simulink model "six_pulse_thyristor_based_rectifier"  (R2026b)
settings: Solver=ode23tb  StopTime=param.sim.simlength  FixedStep=param.glb_time.tc  MaxStep=param.glb_time.tc  EnableMultiTasking=on
values from neighbouring files (symbols this model uses):
  param = struct()    [init_model.m]    (also in init_model_legacy.m = add_template_extras(param, options))
undefined symbols (not defined in the file or in its folder): magnitude
libraries: fl_lib x168, nesl_utility x52, ee_lib x8, thyristor_rr_lib x6, first_harmonic_tracker x3, three_phase_voltage_with_frt_emulator x1
(part 2 of 4)

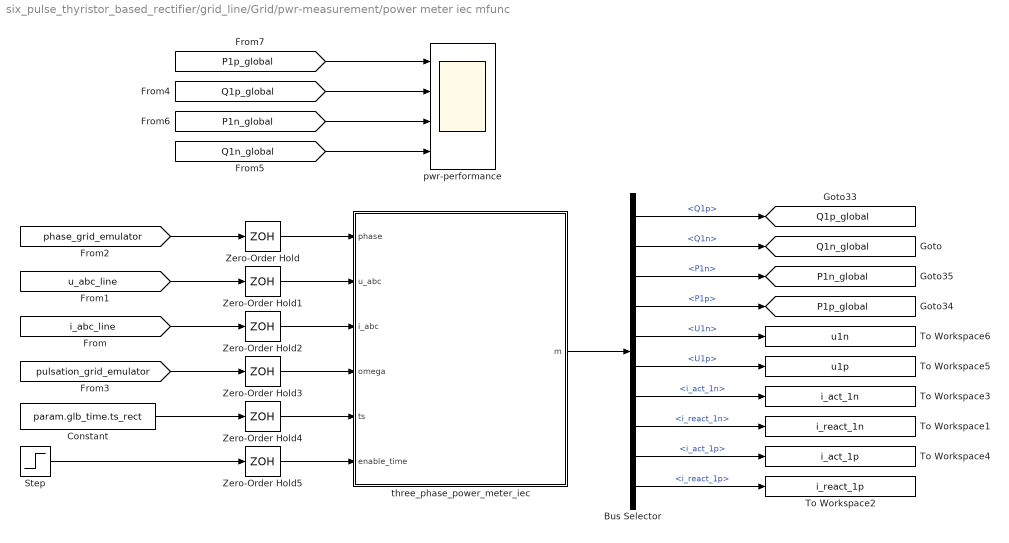
== system six_pulse_thyristor_based_rectifier/grid_line/Grid/pwr-measurement/power meter iec mfunc ==
  Bus Selector : BusSelector  OutputSignals=Q1p,Q1n,P1n,P1p,U1n,U1p,i_act_1n,i_react_1n,i_act_1p,i_react_1p
  Constant : Constant  Value=param.glb_time.ts_rect
  Step : Step  Time=0.025  InitialValue=1  FinalValue=0  SampleTime=0
  To Workspace1 : ToWorkspace  VariableName=i_react_1n  SampleTime=param.glb_time.ts_rect
      settings: MaxDataPoints=param.glb_time.Ns_rect
  To Workspace2 : ToWorkspace  VariableName=i_react_1p  SampleTime=param.glb_time.ts_rect
      settings: MaxDataPoints=param.glb_time.Ns_rect
  To Workspace3 : ToWorkspace  VariableName=i_act_1n  SampleTime=param.glb_time.ts_rect
      settings: MaxDataPoints=param.glb_time.Ns_rect
  To Workspace4 : ToWorkspace  VariableName=i_act_1p  SampleTime=param.glb_time.ts_rect
      settings: MaxDataPoints=param.glb_time.Ns_rect
  To Workspace5 : ToWorkspace  VariableName=u1p  SampleTime=param.glb_time.ts_rect
      settings: MaxDataPoints=param.glb_time.Ns_rect
  To Workspace6 : ToWorkspace  VariableName=u1n  SampleTime=param.glb_time.ts_rect
      settings: MaxDataPoints=param.glb_time.Ns_rect
  Zero-Order Hold{,1..5} (6 alike) : ZeroOrderHold  SampleTime=param.glb_time.ts_rect
  pwr-performance : Scope  NumInputPorts=4
      settings: ActiveDisplayString=4  ActiveDisplayYMinimum=-7285.6137508194915  ActiveDisplayYMaximum=63669.675187339519  DataLoggingVariableName=ScopeData3
  three_phase_power_meter_iec : MATLAB Function  TreatAsAtomicUnit=on  SystemSampleTime=param.glb_time.ts_rect
  tag scope: P1n_global=global, P1p_global=global, Q1n_global=global, Q1p_global=global
  wires:
  Bus Selector/6 -> To Workspace5/1  "<U1p>"
  Bus Selector/8 -> To Workspace1/1  "<i_react_1n>"
  Bus Selector/10 -> To Workspace2/1  "<i_react_1p>"
  Bus Selector/5 -> To Workspace6/1  "<U1n>"
  Bus Selector/4 -> [P1p_global]  "<P1p>"
  Bus Selector/2 -> [Q1n_global]  "<Q1n>"
  Bus Selector/1 -> [Q1p_global]  "<Q1p>"
  Bus Selector/7 -> To Workspace3/1  "<i_act_1n>"
  Bus Selector/9 -> To Workspace4/1  "<i_act_1p>"
  Bus Selector/3 -> [P1n_global]  "<P1n>"
  three_phase_power_meter_iec/1(m) -> Bus Selector/1
  Zero-Order Hold/1 -> three_phase_power_meter_iec/1(phase)
  Zero-Order Hold2/1 -> three_phase_power_meter_iec/3(i_abc)
  [phase_grid_emulator] -> Zero-Order Hold/1
  Step/1 -> Zero-Order Hold5/1
  Zero-Order Hold3/1 -> three_phase_power_meter_iec/4(omega)
  Zero-Order Hold4/1 -> three_phase_power_meter_iec/5(ts)
  [u_abc_line] -> Zero-Order Hold1/1
  Zero-Order Hold5/1 -> three_phase_power_meter_iec/6(enable_time)
  [i_abc_line] -> Zero-Order Hold2/1
  [pulsation_grid_emulator] -> Zero-Order Hold3/1
  Constant/1 -> Zero-Order Hold4/1
  Zero-Order Hold1/1 -> three_phase_power_meter_iec/2(u_abc)
  [Q1p_global] -> pwr-performance/2
  [Q1n_global] -> pwr-performance/4
  [P1n_global] -> pwr-performance/3
  [P1p_global] -> pwr-performance/1

== system six_pulse_thyristor_based_rectifier/grid_line/six_pulse rectifier/BR2/rms ==
  in : Inport
  Gain : Gain  Gain=param.meas.rms.n1-1
  Gain1 : Gain  Gain=1/param.meas.rms.n1
  Math Function : Math  Operator=magnitude^2  SignedPower=on
  Sqrt : Sqrt
  Sum : Sum  Inputs=|++
  Unit Delay : UnitDelay  SampleTime=param.glb_time.tc
  out : Outport  VectorParamsAs1DForOutWhenUnconnected=off
  wires:
  in/1 -> Math Function/1
  Sum/1 -> Gain1/1
  Gain1/1 -> Sqrt/1, Unit Delay/1
  Unit Delay/1 -> Gain/1
  Math Function/1 -> Sum/1
  Sqrt/1 -> out/1
  Gain/1 -> Sum/2

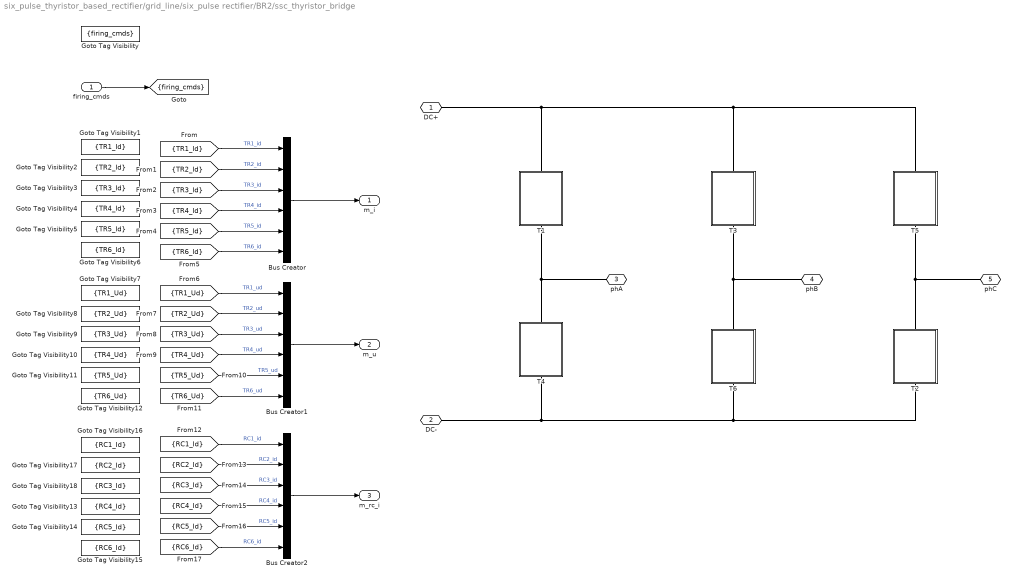
== system six_pulse_thyristor_based_rectifier/grid_line/six_pulse rectifier/BR2/ssc_thyristor_bridge ==
  firing_cmds : Inport
  Bus Creator : BusCreator  Inputs=6
  Bus Creator1 : BusCreator  Inputs=6
  Bus Creator2 : BusCreator  Inputs=6
  Goto Tag Visibility : GotoTagVisibility  GotoTag=firing_cmds
  Goto Tag Visibility1 : GotoTagVisibility  GotoTag=TR1_Id
  Goto Tag Visibility10 : GotoTagVisibility  GotoTag=TR4_Ud
  Goto Tag Visibility11 : GotoTagVisibility  GotoTag=TR5_Ud
  Goto Tag Visibility12 : GotoTagVisibility  GotoTag=TR6_Ud
  Goto Tag Visibility13 : GotoTagVisibility  GotoTag=RC4_Id
  Goto Tag Visibility14 : GotoTagVisibility  GotoTag=RC5_Id
  Goto Tag Visibility15 : GotoTagVisibility  GotoTag=RC6_Id
  Goto Tag Visibility16 : GotoTagVisibility  GotoTag=RC1_Id
  Goto Tag Visibility17 : GotoTagVisibility  GotoTag=RC2_Id
  Goto Tag Visibility18 : GotoTagVisibility  GotoTag=RC3_Id
  Goto Tag Visibility2 : GotoTagVisibility  GotoTag=TR2_Id
  Goto Tag Visibility3 : GotoTagVisibility  GotoTag=TR3_Id
  Goto Tag Visibility4 : GotoTagVisibility  GotoTag=TR4_Id
  Goto Tag Visibility5 : GotoTagVisibility  GotoTag=TR5_Id
  Goto Tag Visibility6 : GotoTagVisibility  GotoTag=TR6_Id
  Goto Tag Visibility7 : GotoTagVisibility  GotoTag=TR1_Ud
  Goto Tag Visibility8 : GotoTagVisibility  GotoTag=TR2_Ud
  Goto Tag Visibility9 : GotoTagVisibility  GotoTag=TR3_Ud
  T1 : Subsystem
  T2 : Subsystem
  T3 : Subsystem
  T4 : Subsystem
  T5 : Subsystem
  T6 : Subsystem
  DC+ : PMIOPort  Side=Left
  DC- : PMIOPort  Port=2  Side=Left
  phA : PMIOPort  Port=3  Side=Right
  phB : PMIOPort  Port=4  Side=Right
  phC : PMIOPort  Port=5  Side=Right
  m_i : Outport
  m_u : Outport  Port=2
  m_rc_i : Outport  Port=3
  tag scope: firing_cmds=scoped
  wires:
  Bus Creator/1 -> m_i/1
  [TR1_Id] -> Bus Creator/1  "TR1_id"
  [TR2_Id] -> Bus Creator/2  "TR2_id"
  [TR3_Id] -> Bus Creator/3  "TR3_id"
  [TR4_Id] -> Bus Creator/4  "TR4_id"
  [TR5_Id] -> Bus Creator/5  "TR5_id"
  [TR6_Id] -> Bus Creator/6  "TR6_id"
  firing_cmds/1 -> [firing_cmds]
  Bus Creator1/1 -> m_u/1
  [TR1_Ud] -> Bus Creator1/1  "TR1_ud"
  [TR2_Ud] -> Bus Creator1/2  "TR2_ud"
  [TR3_Ud] -> Bus Creator1/3  "TR3_ud"
  [TR4_Ud] -> Bus Creator1/4  "TR4_ud"
  [TR5_Ud] -> Bus Creator1/5  "TR5_ud"
  [TR6_Ud] -> Bus Creator1/6  "TR6_ud"
  [RC1_Id] -> Bus Creator2/1  "RC1_id"
  Bus Creator2/1 -> m_rc_i/1
  [RC2_Id] -> Bus Creator2/2  "RC2_id"
  [RC3_Id] -> Bus Creator2/3  "RC3_id"
  [RC4_Id] -> Bus Creator2/4  "RC4_id"
  [RC5_Id] -> Bus Creator2/5  "RC5_id"
  [RC6_Id] -> Bus Creator2/6  "RC6_id"
  connections:
  DC+/RConn1 -- T1/RConn1 -- T3/RConn1 -- T5/RConn1
  T4/RConn1 -- phA/RConn1 -- T1/LConn1
  phC/RConn1 -- T5/LConn1 -- T2/RConn1
  T6/RConn1 -- phB/RConn1 -- T3/LConn1
  T6/LConn1 -- T2/LConn1 -- T4/LConn1 -- DC-/RConn1

== system six_pulse_thyristor_based_rectifier/grid_line/six_pulse rectifier/C-caller ctrl/shift_level ==
  "PY " : Inport
  Bus Selector : BusSelector  OutputSignals=p1,p2,p3,p4,p5,p6
  Data Type Conversion{,1..5} (6 alike) : DataTypeConversion  OutDataTypeStr=double  SaturateOnIntegerOverflow=off  RndMeth=Floor
  Gain{,1..5} (6 alike) : Gain  Gain=param.rect.gate.u_on
  Mux : Mux  Inputs=6
  PY : Outport
  wires:
  Bus Selector/5 -> Data Type Conversion4/1  "<p5>"
  Bus Selector/2 -> Data Type Conversion1/1  "<p2>"
  "PY "/1 -> Bus Selector/1
  Bus Selector/4 -> Data Type Conversion3/1  "<p4>"
  Bus Selector/1 -> Data Type Conversion/1  "<p1>"
  Bus Selector/6 -> Data Type Conversion5/1  "<p6>"
  Mux/1 -> PY/1
  Bus Selector/3 -> Data Type Conversion2/1  "<p3>"
  Data Type Conversion/1 -> Gain/1
  Data Type Conversion1/1 -> Gain1/1
  Data Type Conversion2/1 -> Gain2/1
  Data Type Conversion3/1 -> Gain3/1
  Data Type Conversion4/1 -> Gain4/1
  Data Type Conversion5/1 -> Gain5/1
  Gain/1 -> Mux/1
  Gain1/1 -> Mux/2
  Gain2/1 -> Mux/3
  Gain3/1 -> Mux/4
  Gain4/1 -> Mux/5
  Gain5/1 -> Mux/6

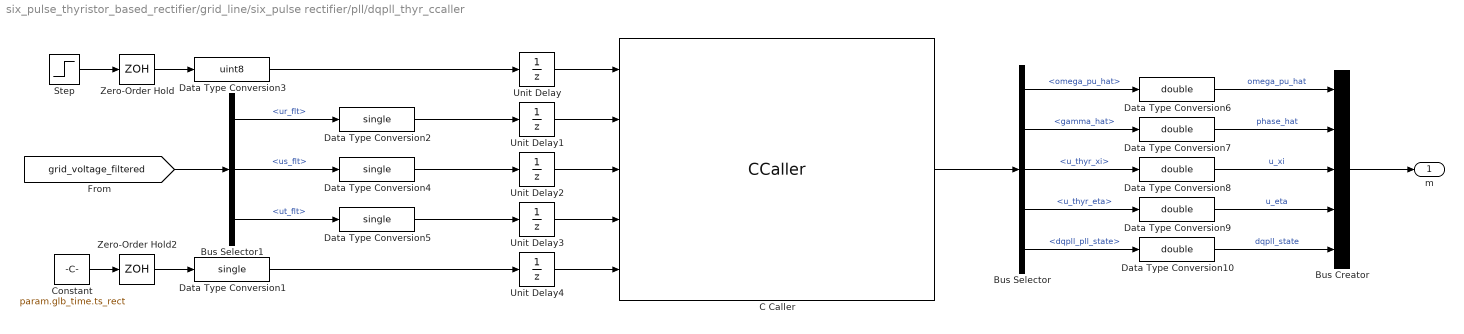
== system six_pulse_thyristor_based_rectifier/grid_line/six_pulse rectifier/pll/dqpll_thyr_ccaller ==
  Bus Creator : BusCreator  Inputs=5
  Bus Selector : BusSelector  OutputSignals=omega_pu_hat,gamma_hat,u_thyr_xi,u_thyr_eta,dqpll_pll_state
  Bus Selector1 : BusSelector  OutputSignals=ur_flt,us_flt,ut_flt
  C Caller : CCaller  FunctionName=dqpll_thyr_process_simulink  PortSpecificationStruct="%)30     .    N H   8    (     @         %    \"     8    !     0         %  0 \"0    $    _    07)G3F%M90  4&]R=$YA;64 4V-O<&4     26YD97@     5'EP90      4VEZ90      27-';&]B86P   X    P    !@    @    $          4    (     0    ,    !         !   P!O=70 #@   #     &    \"     0         !0    @    !     P    $         $  # &]U=  .    .     8    (    !          %    \"     $    &     0         0   ...(+3319 chars)"  SampleTime=param.glb_time.ts_rect
  Constant : Constant  Value=param.glb_time.ts_rect
  Data Type Conversion{1..2,4..5} (4 alike) : DataTypeConversion  OutDataTypeStr=single  SaturateOnIntegerOverflow=off  RndMeth=Floor
  Data Type Conversion{6..10} (5 alike) : DataTypeConversion  OutDataTypeStr=double  SaturateOnIntegerOverflow=off  RndMeth=Floor
  Data Type Conversion3 : DataTypeConversion  OutDataTypeStr=uint8  SaturateOnIntegerOverflow=off  RndMeth=Floor
  Step : Step  Time=param.rect.ctrl.t_pll_reset  InitialValue=1  FinalValue=0  SampleTime=0
  Unit Delay{,1..4} (5 alike) : UnitDelay  SampleTime=param.glb_time.ts_rect
  Zero-Order Hold : ZeroOrderHold  SampleTime=param.glb_time.ts_rect
  Zero-Order Hold2 : ZeroOrderHold  SampleTime=param.glb_time.ts_rect
  m : Outport
  wires:
  Zero-Order Hold/1 -> Data Type Conversion3/1
  Step/1 -> Zero-Order Hold/1
  Zero-Order Hold2/1 -> Data Type Conversion1/1
  Constant/1 -> Zero-Order Hold2/1
  Data Type Conversion3/1 -> Unit Delay/1
  Data Type Conversion2/1 -> Unit Delay1/1
  Data Type Conversion4/1 -> Unit Delay2/1
  Data Type Conversion5/1 -> Unit Delay3/1
  Data Type Conversion1/1 -> Unit Delay4/1
  C Caller/1 -> Bus Selector/1
  Bus Selector/1 -> Data Type Conversion6/1  "<omega_pu_hat>"
  Bus Selector/2 -> Data Type Conversion7/1  "<gamma_hat>"
  Bus Selector/3 -> Data Type Conversion8/1  "<u_thyr_xi>"
  Bus Selector/4 -> Data Type Conversion9/1  "<u_thyr_eta>"
  Bus Selector/5 -> Data Type Conversion10/1  "<dqpll_pll_state>"
  Data Type Conversion6/1 -> Bus Creator/1  "omega_pu_hat"
  Data Type Conversion7/1 -> Bus Creator/2  "phase_hat"
  Data Type Conversion10/1 -> Bus Creator/5  "dqpll_state"
  Data Type Conversion8/1 -> Bus Creator/3  "u_xi"
  Data Type Conversion9/1 -> Bus Creator/4  "u_eta"
  [grid_voltage_filtered] -> Bus Selector1/1
  Unit Delay/1 -> C Caller/1
  Unit Delay1/1 -> C Caller/2
  Unit Delay2/1 -> C Caller/3
  Unit Delay3/1 -> C Caller/4
  Unit Delay4/1 -> C Caller/5
  Bus Creator/1 -> m/1
  Bus Selector1/1 -> Data Type Conversion2/1  "<ur_flt>"
  Bus Selector1/2 -> Data Type Conversion4/1  "<us_flt>"
  Bus Selector1/3 -> Data Type Conversion5/1  "<ut_flt>"

== system six_pulse_thyristor_based_rectifier/grid_line/six_pulse rectifier/pll/pll_stageA ==
  ug : Inport
  Demux : Demux  Outputs=3
  Math Function : Math  Operator=magnitude^2  SignedPower=on
  Math Function1 : Math  Operator=magnitude^2  SignedPower=on
  Reciprocal Sqrt : Sqrt  Operator=rSqrt
  Saturation : Saturate  UpperLimit=inf  LowerLimit=0.001
  Sum : Sum  Inputs=|++
  abc2alphabeta : Subsystem
  Vgrid_a : Outport
  Vgrid_b : Outport  Port=2
  tag scope: Vgrid_unorm_posneg=global
  wires:
  ug/1 -> Demux/1
  Demux/1 -> abc2alphabeta/1(Vgrid_a)
  Demux/2 -> abc2alphabeta/2(Vgrid_b)
  Demux/3 -> abc2alphabeta/3(Vgrid_c)
  abc2alphabeta/1(Vgrid_alpha) -> Vgrid_a/1, Math Function/1
  abc2alphabeta/2(Vgrid_beta) -> Math Function1/1, Vgrid_b/1
  Math Function/1 -> Sum/1
  Math Function1/1 -> Sum/2
  Sum/1 -> Saturation/1
  Reciprocal Sqrt/1 -> [Vgrid_unorm_posneg]
  Saturation/1 -> Reciprocal Sqrt/1

== system six_pulse_thyristor_based_rectifier/grid_line/six_pulse rectifier/pll/pll_stageB ==
  Vgrid_a : Inport
  Vgrid_b : Inport  Port=2
  Unit Delay2 : UnitDelay  SampleTime=param.glb_time.ts_rect
  alphabeta2xieta : Subsystem
  pll_2 : Subsystem
  wt_grid : Outport
  wires:
  Vgrid_a/1 -> alphabeta2xieta/1(alpha)
  Vgrid_b/1 -> alphabeta2xieta/2(beta)
  Unit Delay2/1 -> alphabeta2xieta/3(wt), wt_grid/1
  pll_2/1(theta_est) -> Unit Delay2/1
  alphabeta2xieta/2(eta) -> pll_2/1(eta)

== system six_pulse_thyristor_based_rectifier/grid_line/six_pulse rectifier/BR2/ssc_thyristor_bridge/T1 ==
  Thyristor_1 : Subsystem
      settings: PortSchema="{\"entries\":[{\"content\":{\"sides\":[{\"content\":{},\"type\":\"ConnectorPlacement.EquallySpacedRectSide\",\"uuid\":\"7269b907-ab9b-4481-ac18-a8dd984c3818\"},{\"content\":{\"connectorIds\":[\"RConn1\"],\"side\":\"RIGHT\"},\"type\":\"ConnectorPlacement.EquallySpacedRectSide\",\"uuid\":\"8dceca02-62a3-4342-b624-c7d4418298d0\"},{\"content\":{\"connectorIds\":[\"LConn1\"],\"side\":\"TOP\"},\"type\":\"ConnectorPlacement.EquallySpacedRectSide\",\"uuid\":\"a3401fa4-31f5-4c91-8a09-9f2730c54d6f\"},{\"content\":{\"connectorIds\":[\"RConn2\"],\"side\":\"BOTTOM\"},\"type\":\"ConnectorPlacement.EquallySpacedRectSide\",\"uuid\":\"ec3e6ca2-4822-4b63-8ee1-1049d14efe1d\"}]},\"type\":\"ConnectorPlacement.EquallySpacedConnector\",\"uuid\":\"06f44f8b-bef4-44e1-af36-23832e4d595a\"}],\"packageUris\":[\"http://schema.mathworks.com/mf0/Connector/R2020b\"],\"version\":\"1.0\"}"
  firing1 : Subsystem
  K : PMIOPort  Side=Right
  A : PMIOPort  Port=2  Side=Left
  connections:
  Thyristor_1/LConn1 -- K/RConn1
  Thyristor_1/RConn1 -- firing1/RConn1
  A/RConn1 -- Thyristor_1/RConn2

== system six_pulse_thyristor_based_rectifier/grid_line/six_pulse rectifier/BR2/ssc_thyristor_bridge/T2 ==
  Thyristor_2 : Subsystem
      settings: PortSchema="{\"entries\":[{\"content\":{\"sides\":[{\"content\":{},\"type\":\"ConnectorPlacement.EquallySpacedRectSide\",\"uuid\":\"7269b907-ab9b-4481-ac18-a8dd984c3818\"},{\"content\":{\"connectorIds\":[\"RConn1\"],\"side\":\"RIGHT\"},\"type\":\"ConnectorPlacement.EquallySpacedRectSide\",\"uuid\":\"8dceca02-62a3-4342-b624-c7d4418298d0\"},{\"content\":{\"connectorIds\":[\"LConn1\"],\"side\":\"TOP\"},\"type\":\"ConnectorPlacement.EquallySpacedRectSide\",\"uuid\":\"a3401fa4-31f5-4c91-8a09-9f2730c54d6f\"},{\"content\":{\"connectorIds\":[\"RConn2\"],\"side\":\"BOTTOM\"},\"type\":\"ConnectorPlacement.EquallySpacedRectSide\",\"uuid\":\"ec3e6ca2-4822-4b63-8ee1-1049d14efe1d\"}]},\"type\":\"ConnectorPlacement.EquallySpacedConnector\",\"uuid\":\"06f44f8b-bef4-44e1-af36-23832e4d595a\"}],\"packageUris\":[\"http://schema.mathworks.com/mf0/Connector/R2020b\"],\"version\":\"1.0\"}"
  firing2 : Subsystem
  K : PMIOPort  Side=Right
  A : PMIOPort  Port=2  Side=Left
  connections:
  Thyristor_2/RConn2 -- A/RConn1
  Thyristor_2/LConn1 -- K/RConn1
  firing2/RConn1 -- Thyristor_2/RConn1

== system six_pulse_thyristor_based_rectifier/grid_line/six_pulse rectifier/BR2/ssc_thyristor_bridge/T3 ==
  Thyristor_3 : Subsystem
      settings: PortSchema="{\"entries\":[{\"content\":{\"sides\":[{\"content\":{},\"type\":\"ConnectorPlacement.EquallySpacedRectSide\",\"uuid\":\"7269b907-ab9b-4481-ac18-a8dd984c3818\"},{\"content\":{\"connectorIds\":[\"RConn1\"],\"side\":\"RIGHT\"},\"type\":\"ConnectorPlacement.EquallySpacedRectSide\",\"uuid\":\"8dceca02-62a3-4342-b624-c7d4418298d0\"},{\"content\":{\"connectorIds\":[\"LConn1\"],\"side\":\"TOP\"},\"type\":\"ConnectorPlacement.EquallySpacedRectSide\",\"uuid\":\"a3401fa4-31f5-4c91-8a09-9f2730c54d6f\"},{\"content\":{\"connectorIds\":[\"RConn2\"],\"side\":\"BOTTOM\"},\"type\":\"ConnectorPlacement.EquallySpacedRectSide\",\"uuid\":\"ec3e6ca2-4822-4b63-8ee1-1049d14efe1d\"}]},\"type\":\"ConnectorPlacement.EquallySpacedConnector\",\"uuid\":\"06f44f8b-bef4-44e1-af36-23832e4d595a\"}],\"packageUris\":[\"http://schema.mathworks.com/mf0/Connector/R2020b\"],\"version\":\"1.0\"}"
  firing3 : Subsystem
  K : PMIOPort  Side=Right
  A : PMIOPort  Port=2  Side=Left
  connections:
  A/RConn1 -- Thyristor_3/RConn2
  Thyristor_3/LConn1 -- K/RConn1
  firing3/RConn1 -- Thyristor_3/RConn1

== system six_pulse_thyristor_based_rectifier/grid_line/six_pulse rectifier/BR2/ssc_thyristor_bridge/T4 ==
  Thyristor_4 : Subsystem
      settings: PortSchema="{\"entries\":[{\"content\":{\"sides\":[{\"content\":{},\"type\":\"ConnectorPlacement.EquallySpacedRectSide\",\"uuid\":\"7269b907-ab9b-4481-ac18-a8dd984c3818\"},{\"content\":{\"connectorIds\":[\"RConn1\"],\"side\":\"RIGHT\"},\"type\":\"ConnectorPlacement.EquallySpacedRectSide\",\"uuid\":\"8dceca02-62a3-4342-b624-c7d4418298d0\"},{\"content\":{\"connectorIds\":[\"LConn1\"],\"side\":\"TOP\"},\"type\":\"ConnectorPlacement.EquallySpacedRectSide\",\"uuid\":\"a3401fa4-31f5-4c91-8a09-9f2730c54d6f\"},{\"content\":{\"connectorIds\":[\"RConn2\"],\"side\":\"BOTTOM\"},\"type\":\"ConnectorPlacement.EquallySpacedRectSide\",\"uuid\":\"ec3e6ca2-4822-4b63-8ee1-1049d14efe1d\"}]},\"type\":\"ConnectorPlacement.EquallySpacedConnector\",\"uuid\":\"06f44f8b-bef4-44e1-af36-23832e4d595a\"}],\"packageUris\":[\"http://schema.mathworks.com/mf0/Connector/R2020b\"],\"version\":\"1.0\"}"
  firing4 : Subsystem
  K : PMIOPort  Side=Right
  A : PMIOPort  Port=2  Side=Left
  connections:
  A/RConn1 -- Thyristor_4/RConn2
  Thyristor_4/LConn1 -- K/RConn1
  firing4/RConn1 -- Thyristor_4/RConn1

== system six_pulse_thyristor_based_rectifier/grid_line/six_pulse rectifier/BR2/ssc_thyristor_bridge/T5 ==
  Thyristor_5 : Subsystem
      settings: PortSchema="{\"entries\":[{\"content\":{\"sides\":[{\"content\":{},\"type\":\"ConnectorPlacement.EquallySpacedRectSide\",\"uuid\":\"7269b907-ab9b-4481-ac18-a8dd984c3818\"},{\"content\":{\"connectorIds\":[\"RConn1\"],\"side\":\"RIGHT\"},\"type\":\"ConnectorPlacement.EquallySpacedRectSide\",\"uuid\":\"8dceca02-62a3-4342-b624-c7d4418298d0\"},{\"content\":{\"connectorIds\":[\"LConn1\"],\"side\":\"TOP\"},\"type\":\"ConnectorPlacement.EquallySpacedRectSide\",\"uuid\":\"a3401fa4-31f5-4c91-8a09-9f2730c54d6f\"},{\"content\":{\"connectorIds\":[\"RConn2\"],\"side\":\"BOTTOM\"},\"type\":\"ConnectorPlacement.EquallySpacedRectSide\",\"uuid\":\"ec3e6ca2-4822-4b63-8ee1-1049d14efe1d\"}]},\"type\":\"ConnectorPlacement.EquallySpacedConnector\",\"uuid\":\"06f44f8b-bef4-44e1-af36-23832e4d595a\"}],\"packageUris\":[\"http://schema.mathworks.com/mf0/Connector/R2020b\"],\"version\":\"1.0\"}"
  firing5 : Subsystem
  K : PMIOPort  Side=Right
  A : PMIOPort  Port=2  Side=Left
  connections:
  Thyristor_5/RConn2 -- A/RConn1
  Thyristor_5/LConn1 -- K/RConn1
  firing5/RConn1 -- Thyristor_5/RConn1

== system six_pulse_thyristor_based_rectifier/grid_line/six_pulse rectifier/BR2/ssc_thyristor_bridge/T6 ==
  Thyristor_6 : Subsystem
      settings: PortSchema="{\"entries\":[{\"content\":{\"sides\":[{\"content\":{},\"type\":\"ConnectorPlacement.EquallySpacedRectSide\",\"uuid\":\"7269b907-ab9b-4481-ac18-a8dd984c3818\"},{\"content\":{\"connectorIds\":[\"RConn1\"],\"side\":\"RIGHT\"},\"type\":\"ConnectorPlacement.EquallySpacedRectSide\",\"uuid\":\"8dceca02-62a3-4342-b624-c7d4418298d0\"},{\"content\":{\"connectorIds\":[\"LConn1\"],\"side\":\"TOP\"},\"type\":\"ConnectorPlacement.EquallySpacedRectSide\",\"uuid\":\"a3401fa4-31f5-4c91-8a09-9f2730c54d6f\"},{\"content\":{\"connectorIds\":[\"RConn2\"],\"side\":\"BOTTOM\"},\"type\":\"ConnectorPlacement.EquallySpacedRectSide\",\"uuid\":\"ec3e6ca2-4822-4b63-8ee1-1049d14efe1d\"}]},\"type\":\"ConnectorPlacement.EquallySpacedConnector\",\"uuid\":\"06f44f8b-bef4-44e1-af36-23832e4d595a\"}],\"packageUris\":[\"http://schema.mathworks.com/mf0/Connector/R2020b\"],\"version\":\"1.0\"}"
  firing6 : Subsystem
  K : PMIOPort  Side=Right
  A : PMIOPort  Port=2  Side=Left
  connections:
  Thyristor_6/LConn1 -- K/RConn1
  A/RConn1 -- Thyristor_6/RConn2
  firing6/RConn1 -- Thyristor_6/RConn1

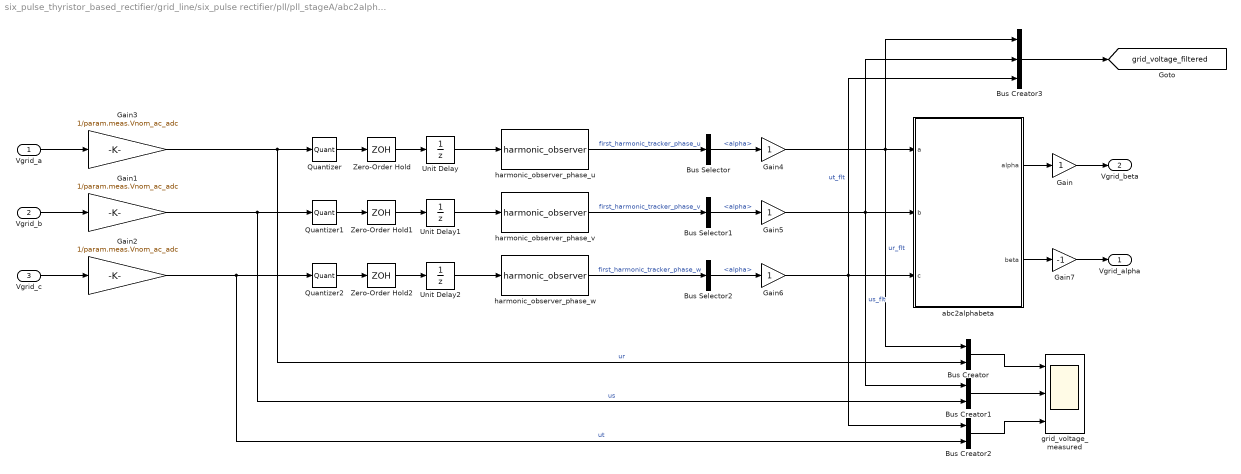
== system six_pulse_thyristor_based_rectifier/grid_line/six_pulse rectifier/pll/pll_stageA/abc2alphabeta ==
  Vgrid_a : Inport
  Vgrid_b : Inport  Port=2
  Vgrid_c : Inport  Port=3
  Bus Creator : BusCreator  Inputs=2
  Bus Creator1 : BusCreator  Inputs=2
  Bus Creator2 : BusCreator  Inputs=2
  Bus Creator3 : BusCreator  Inputs=3
  Bus Selector : BusSelector  OutputSignals=alpha
  Bus Selector1 : BusSelector  OutputSignals=alpha
  Bus Selector2 : BusSelector  OutputSignals=alpha
  Gain{,4..6} (4 alike) : Gain
  Gain1 : Gain  Gain=1/param.meas.Vnom_ac_adc
  Gain2 : Gain  Gain=1/param.meas.Vnom_ac_adc
  Gain3 : Gain  Gain=1/param.meas.Vnom_ac_adc
  Gain7 : Gain  Gain=-1
  Quantizer : Quantizer  QuantizationInterval=2^-11
  Quantizer1 : Quantizer  QuantizationInterval=2^-11
  Quantizer2 : Quantizer  QuantizationInterval=2^-11
  Unit Delay : UnitDelay  SampleTime=param.glb_time.ts_rect
  Unit Delay1 : UnitDelay  SampleTime=param.glb_time.ts_rect
  Unit Delay2 : UnitDelay  SampleTime=param.glb_time.ts_rect
  Zero-Order Hold : ZeroOrderHold  SampleTime=param.glb_time.ts_rect
  Zero-Order Hold1 : ZeroOrderHold  SampleTime=param.glb_time.ts_rect
  Zero-Order Hold2 : ZeroOrderHold  SampleTime=param.glb_time.ts_rect
  abc2alphabeta : Subsystem
  grid_voltage_measured : Scope  NumInputPorts=3
      settings: ActiveDisplayYMinimum=-2.4352832318691768  ActiveDisplayYMaximum=1.5799082777235063
  harmonic_observer_phase_u : first_harmonic_tracker/harmonic_observer  omega_base=param.rect.ctrl.fht.omega_base  delta=param.rect.ctrl.fht.delta  pole1=param.rect.ctrl.fht.pole1  pole2=param.rect.ctrl.fht.pole2  ts=param.glb_time.ts_rect
  harmonic_observer_phase_v : first_harmonic_tracker/harmonic_observer  omega_base=param.rect.ctrl.fht.omega_base  delta=param.rect.ctrl.fht.delta  pole1=param.rect.ctrl.fht.pole1  pole2=param.rect.ctrl.fht.pole2  ts=param.glb_time.ts_rect
  harmonic_observer_phase_w : first_harmonic_tracker/harmonic_observer  omega_base=param.rect.ctrl.fht.omega_base  delta=param.rect.ctrl.fht.delta  pole1=param.rect.ctrl.fht.pole1  pole2=param.rect.ctrl.fht.pole2  ts=param.glb_time.ts_rect
  Vgrid_alpha : Outport
  Vgrid_beta : Outport  Port=2
  tag scope: grid_voltage_filtered=global
  wires:
  Vgrid_a/1 -> Gain3/1
  abc2alphabeta/2("beta ") -> Gain7/1
  abc2alphabeta/1("alpha ") -> Gain/1
  Gain/1 -> Vgrid_beta/1
  Gain7/1 -> Vgrid_alpha/1
  Zero-Order Hold/1 -> Unit Delay/1
  Bus Creator3/1 -> [grid_voltage_filtered]
  Bus Creator/1 -> grid_voltage_measured/1
  Bus Creator1/1 -> grid_voltage_measured/2
  Bus Creator2/1 -> grid_voltage_measured/3
  Bus Selector/1 -> Gain4/1  "<alpha>"
  Unit Delay/1 -> harmonic_observer_phase_u/1
  Quantizer2/1 -> Zero-Order Hold2/1
  Gain3/1 -> Quantizer/1, Bus Creator/2  "ur"
  Vgrid_b/1 -> Gain1/1
  Vgrid_c/1 -> Gain2/1
  Quantizer/1 -> Zero-Order Hold/1
  Quantizer1/1 -> Zero-Order Hold1/1
  Unit Delay1/1 -> harmonic_observer_phase_v/1
  Unit Delay2/1 -> harmonic_observer_phase_w/1
  Zero-Order Hold1/1 -> Unit Delay1/1
  Zero-Order Hold2/1 -> Unit Delay2/1
  Gain1/1 -> Quantizer1/1, Bus Creator1/2  "us"
  Gain2/1 -> Quantizer2/1, Bus Creator2/2  "ut"
  harmonic_observer_phase_u/1 -> Bus Selector/1  "first_harmonic_tracker_phase_u"
  harmonic_observer_phase_v/1 -> Bus Selector1/1  "first_harmonic_tracker_phase_v"
  Bus Selector1/1 -> Gain5/1  "<alpha>"
  harmonic_observer_phase_w/1 -> Bus Selector2/1  "first_harmonic_tracker_phase_w"
  Bus Selector2/1 -> Gain6/1  "<alpha>"
  Gain4/1 -> Bus Creator/1, Bus Creator3/1, abc2alphabeta/1(a)  "ur_flt"
  Gain5/1 -> Bus Creator3/2, Bus Creator1/1, abc2alphabeta/2(b)  "us_flt"
  Gain6/1 -> Bus Creator3/3, Bus Creator2/1, abc2alphabeta/3(c)  "ut_flt"

== system six_pulse_thyristor_based_rectifier/grid_line/six_pulse rectifier/pll/pll_stageB/alphabeta2xieta ==
  alpha : Inport
  beta : Inport  Port=2
  wt : Inport  Port=3
  Product{,1..3} (4 alike) : Product  RndMeth=Zero
  Sum : Sum
  Sum1 : Sum  Inputs=-+
  Trigonometric Function : Trigonometry  Operator=cos
  Trigonometric Function1 : Trigonometry
  xi : Outport
  eta : Outport  Port=2
  wires:
  Trigonometric Function/1 -> [cos]
  Trigonometric Function1/1 -> [sin]
  wt/1 -> Trigonometric Function1/1, Trigonometric Function/1
  Sum1/1 -> eta/1
  Sum/1 -> xi/1
  [cos] -> Product3/1
  Product3/1 -> Sum1/2
  Product2/1 -> Sum1/1
  [sin] -> Product2/1
  beta/1 -> Product3/2, Product1/2
  [sin] -> Product1/1
  Product1/1 -> Sum/2
  Product/1 -> Sum/1
  alpha/1 -> Product2/2, Product/2
  [cos] -> Product/1

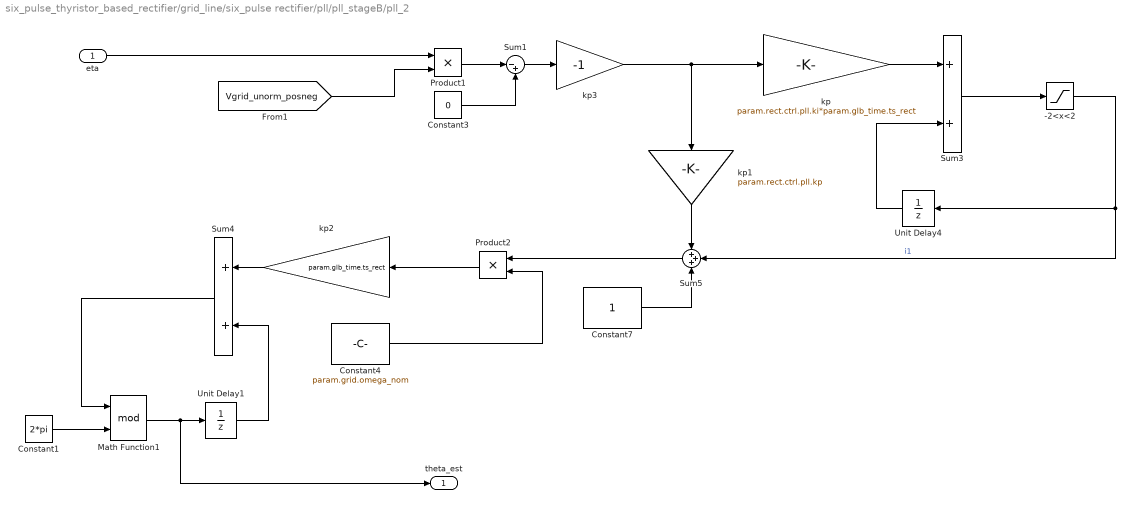
== system six_pulse_thyristor_based_rectifier/grid_line/six_pulse rectifier/pll/pll_stageB/pll_2 ==
  eta : Inport
  -2<x<2 : Saturate  UpperLimit=2  LowerLimit=-2
  Constant1 : Constant  Value=2*pi
  Constant3 : Constant  Value=0
  Constant4 : Constant  Value=param.grid.omega_nom
  Constant7 : Constant
  Math Function1 : Math  Operator=mod  SignedPower=on
  Product1 : Product  RndMeth=Zero
  Product2 : Product  RndMeth=Zero
  Sum1 : Sum  Inputs=|-+
  Sum3 : Sum  SaturateOnIntegerOverflow=on
  Sum4 : Sum  SaturateOnIntegerOverflow=on
  Sum5 : Sum  Inputs=+++
  Unit Delay1 : UnitDelay  SampleTime=param.glb_time.ts_rect
  Unit Delay4 : UnitDelay  SampleTime=param.glb_time.ts_rect
  kp : Gain  Gain=param.rect.ctrl.pll.ki*param.glb_time.ts_rect  SaturateOnIntegerOverflow=on  OutDataTypeStr=Inherit: Same as input  ParamDataTypeStr=Inherit: Same as input
  kp1 : Gain  Gain=param.rect.ctrl.pll.kp  SaturateOnIntegerOverflow=on  OutDataTypeStr=Inherit: Same as input  ParamDataTypeStr=Inherit: Same as input
  kp2 : Gain  Gain=param.glb_time.ts_rect  SaturateOnIntegerOverflow=on  OutDataTypeStr=Inherit: Same as input  ParamDataTypeStr=Inherit: Same as input
  kp3 : Gain  Gain=-1  SaturateOnIntegerOverflow=on  OutDataTypeStr=Inherit: Same as input  ParamDataTypeStr=Inherit: Same as input
  theta_est : Outport
  wires:
  Constant7/1 -> Sum5/3
  Constant3/1 -> Sum1/2
  [Vgrid_unorm_posneg] -> Product1/2
  Product2/1 -> kp2/1
  kp/1 -> Sum3/1
  Sum4/1 -> Math Function1/1
  kp1/1 -> Sum5/1
  Product1/1 -> Sum1/1
  Sum1/1 -> kp3/1
  Math Function1/1 -> theta_est/1, Unit Delay1/1
  -2<x<2/1 -> Unit Delay4/1, Sum5/2  "i1"
  Unit Delay4/1 -> Sum3/2
  Sum3/1 -> -2<x<2/1
  kp2/1 -> Sum4/1
  Sum5/1 -> Product2/1
  Constant4/1 -> Product2/2
  Unit Delay1/1 -> Sum4/2
  Constant1/1 -> Math Function1/2
  eta/1 -> Product1/1
  kp3/1 -> kp/1, kp1/1

== system six_pulse_thyristor_based_rectifier/grid_line/six_pulse rectifier/BR2/ssc_thyristor_bridge/T1/Thyristor_1 ==
  Capacitor : fl_lib/Electrical/Electrical Elements/Capacitor  c=Csnubber_m F  r=Rsnubber_m Ohm  g=0 1/Ohm  i_specify=off  i_priority=None  i=0 A  i_nominal_specify=off  i_nominal_value=1  i_nominal_unit=A  v_specify=off  v_priority=None  v=0 V  v_nominal_specify=off  v_nominal_value=1  v_nominal_unit=V  vc_specify=off  vc_priority=High  vc=0 V  vc_nominal_specify=off  vc_nominal_value=1  vc_nominal_unit=V
  Current Sensor : fl_lib/Electrical/Electrical Sensors/Current Sensor
  Current Sensor1 : fl_lib/Electrical/Electrical Sensors/Current Sensor
  PS-Simulink Converter : nesl_utility/PS-Simulink Converter  PhysicalDomain=network_engine_domain  SubClassName=ps_output  LeftPortType=input  RightPortType=output  PseudoPeriodic=off  Frequencies=[]  VectorFormat=1-D array  Unit=A  AffineConversion=off
  PS-Simulink Converter1 : nesl_utility/PS-Simulink Converter  PhysicalDomain=network_engine_domain  SubClassName=ps_output  LeftPortType=input  RightPortType=output  PseudoPeriodic=off  Frequencies=[]  VectorFormat=1-D array  Unit=V  AffineConversion=off
  PS-Simulink Converter2 : nesl_utility/PS-Simulink Converter  PhysicalDomain=network_engine_domain  SubClassName=ps_output  LeftPortType=input  RightPortType=output  PseudoPeriodic=off  Frequencies=[]  VectorFormat=1-D array  Unit=A  AffineConversion=off
  Thyristor with Reverse Recovery (Lauritzen-Ma charge dynamics) : thyristor_rr_lib/Thyristor with Reverse Recovery (Lauritzen-Ma charge dynamics)  Vf=Vf_m V  Ron=Ron_m Ohm  Goff=Goff_m 1/Ohm  Vgt=Vgt_m V  Vth=forward_voltage_threshold_m V  Il=latching_current_m A  Ih=holding_current_m A  tau=carrier_lifetime_m s  Tm=charge_cross_time_constant_m s  Qth=residual_charge_threshold_m C  tq=circuit_commutated_turn_off_time_m s  i_specify=off  i_priority=None  i=0 A  i_nominal_specify=off  i_nominal_value=1  i_nominal_unit=A  v_specify=off  v_priority=None  v=0 V  v_nominal_specify=off  v_nominal_value=1  v_nominal_unit=V  qM_specify=off  qM_priority=High  qM=0 C  qM_nominal_specify=off  qM_nominal_value=1  qM_nominal_unit=C  on_specify=off  on_priority=None  on=0  toff_specify=off  toff_priority=None  toff=-1 s
  Voltage Sensor : fl_lib/Electrical/Electrical Sensors/Voltage Sensor
  K : PMIOPort  Side=Left
  G : PMIOPort  Port=2  Side=Right
  A : PMIOPort  Port=3  Side=Right
  tag scope: RC1_Id=scoped, TR1_Id=scoped, TR1_Ud=scoped
  wires:
  PS-Simulink Converter/1 -> [TR1_Id]
  PS-Simulink Converter2/1 -> [RC1_Id]
  PS-Simulink Converter1/1 -> [TR1_Ud]
  connections:
  K/RConn1 -- Capacitor/LConn1 -- Thyristor with Reverse Recovery (Lauritzen-Ma charge dynamics)/RConn1 -- Voltage Sensor/RConn2
  PS-Simulink Converter1/LConn1 -- Voltage Sensor/RConn1
  PS-Simulink Converter/LConn1 -- Current Sensor/RConn1
  Current Sensor1/RConn2 -- Capacitor/RConn1
  Current Sensor/RConn2 -- Thyristor with Reverse Recovery (Lauritzen-Ma charge dynamics)/LConn1 -- Voltage Sensor/LConn1 -- Current Sensor1/LConn1
  PS-Simulink Converter2/LConn1 -- Current Sensor1/RConn1
  Thyristor with Reverse Recovery (Lauritzen-Ma charge dynamics)/RConn2 -- G/RConn1
  A/RConn1 -- Current Sensor/LConn1

== system six_pulse_thyristor_based_rectifier/grid_line/six_pulse rectifier/BR2/ssc_thyristor_bridge/T1/firing1 ==
  Selector : Selector  InputPortWidth=6  IndexOptions=Index vector (dialog)  Indices=1  OutputSizes=1  RuntimeRangeChecks=off
  Simulink-PS Converter : nesl_utility/Simulink-PS Converter  PhysicalDomain=network_engine_domain  SubClassName=ps_input  LeftPortType=input  RightPortType=output  PseudoPeriodic=off  Frequencies=[]  NoiseDistribution=none  NoiseParameters=[]  Unit=V  AffineConversion=off  FilteringAndDerivatives=provide  SimscapeFilterOrder=1  InputFilterTimeConstant=0.001  UdotUserProvided=0
  firing_circuit : Subsystem
  strobe_gnr : Subsystem  Commented=through
  g+ : PMIOPort  Side=Right
  wires:
  strobe_gnr/1(out) -> Simulink-PS Converter/1
  Selector/1 -> strobe_gnr/1(in)
  [firing_cmds] -> Selector/1
  connections:
  g+/RConn1 -- firing_circuit/RConn1
  Simulink-PS Converter/RConn1 -- firing_circuit/LConn1

== system six_pulse_thyristor_based_rectifier/grid_line/six_pulse rectifier/BR2/ssc_thyristor_bridge/T2/Thyristor_2 ==
  Capacitor : fl_lib/Electrical/Electrical Elements/Capacitor  c=Csnubber_m F  r=Rsnubber_m Ohm  g=0 1/Ohm  i_specify=off  i_priority=None  i=0 A  i_nominal_specify=off  i_nominal_value=1  i_nominal_unit=A  v_specify=off  v_priority=None  v=0 V  v_nominal_specify=off  v_nominal_value=1  v_nominal_unit=V  vc_specify=off  vc_priority=High  vc=0 V  vc_nominal_specify=off  vc_nominal_value=1  vc_nominal_unit=V
  Current Sensor : fl_lib/Electrical/Electrical Sensors/Current Sensor
  Current Sensor1 : fl_lib/Electrical/Electrical Sensors/Current Sensor
  PS-Simulink Converter : nesl_utility/PS-Simulink Converter  PhysicalDomain=network_engine_domain  SubClassName=ps_output  LeftPortType=input  RightPortType=output  PseudoPeriodic=off  Frequencies=[]  VectorFormat=1-D array  Unit=A  AffineConversion=off
  PS-Simulink Converter1 : nesl_utility/PS-Simulink Converter  PhysicalDomain=network_engine_domain  SubClassName=ps_output  LeftPortType=input  RightPortType=output  PseudoPeriodic=off  Frequencies=[]  VectorFormat=1-D array  Unit=V  AffineConversion=off
  PS-Simulink Converter2 : nesl_utility/PS-Simulink Converter  PhysicalDomain=network_engine_domain  SubClassName=ps_output  LeftPortType=input  RightPortType=output  PseudoPeriodic=off  Frequencies=[]  VectorFormat=1-D array  Unit=A  AffineConversion=off
  Thyristor with Reverse Recovery (Lauritzen-Ma charge dynamics) : thyristor_rr_lib/Thyristor with Reverse Recovery (Lauritzen-Ma charge dynamics)  Vf=Vf_m V  Ron=Ron_m Ohm  Goff=Goff_m 1/Ohm  Vgt=Vgt_m V  Vth=forward_voltage_threshold_m V  Il=latching_current_m A  Ih=holding_current_m A  tau=carrier_lifetime_m s  Tm=charge_cross_time_constant_m s  Qth=residual_charge_threshold_m C  tq=circuit_commutated_turn_off_time_m s  i_specify=off  i_priority=None  i=0 A  i_nominal_specify=off  i_nominal_value=1  i_nominal_unit=A  v_specify=off  v_priority=None  v=0 V  v_nominal_specify=off  v_nominal_value=1  v_nominal_unit=V  qM_specify=off  qM_priority=High  qM=0 C  qM_nominal_specify=off  qM_nominal_value=1  qM_nominal_unit=C  on_specify=off  on_priority=None  on=0  toff_specify=off  toff_priority=None  toff=-1 s
  Voltage Sensor : fl_lib/Electrical/Electrical Sensors/Voltage Sensor
  K : PMIOPort  Side=Left
  G : PMIOPort  Port=2  Side=Right
  A : PMIOPort  Port=3  Side=Right
  tag scope: RC2_Id=scoped, TR2_Id=scoped, TR2_Ud=scoped
  wires:
  PS-Simulink Converter/1 -> [TR2_Id]
  PS-Simulink Converter2/1 -> [RC2_Id]
  PS-Simulink Converter1/1 -> [TR2_Ud]
  connections:
  Capacitor/LConn1 -- Voltage Sensor/RConn2 -- Thyristor with Reverse Recovery (Lauritzen-Ma charge dynamics)/RConn1 -- K/RConn1
  PS-Simulink Converter1/LConn1 -- Voltage Sensor/RConn1
  PS-Simulink Converter/LConn1 -- Current Sensor/RConn1
  Current Sensor1/RConn2 -- Capacitor/RConn1
  Voltage Sensor/LConn1 -- Current Sensor1/LConn1 -- Thyristor with Reverse Recovery (Lauritzen-Ma charge dynamics)/LConn1 -- Current Sensor/RConn2
  PS-Simulink Converter2/LConn1 -- Current Sensor1/RConn1
  Thyristor with Reverse Recovery (Lauritzen-Ma charge dynamics)/RConn2 -- G/RConn1
  A/RConn1 -- Current Sensor/LConn1

== system six_pulse_thyristor_based_rectifier/grid_line/six_pulse rectifier/BR2/ssc_thyristor_bridge/T2/firing2 ==
  Selector : Selector  InputPortWidth=6  IndexOptions=Index vector (dialog)  Indices=2  OutputSizes=1  RuntimeRangeChecks=off
  Simulink-PS Converter : nesl_utility/Simulink-PS Converter  PhysicalDomain=network_engine_domain  SubClassName=ps_input  LeftPortType=input  RightPortType=output  PseudoPeriodic=off  Frequencies=[]  NoiseDistribution=none  NoiseParameters=[]  Unit=V  AffineConversion=off  FilteringAndDerivatives=provide  SimscapeFilterOrder=1  InputFilterTimeConstant=0.001  UdotUserProvided=0
  firing_circuit : Subsystem
  strobe_gnr : Subsystem  Commented=through
  g+ : PMIOPort  Side=Right
  wires:
  strobe_gnr/1(out) -> Simulink-PS Converter/1
  Selector/1 -> strobe_gnr/1(in)
  [firing_cmds] -> Selector/1
  connections:
  Simulink-PS Converter/RConn1 -- firing_circuit/LConn1
  g+/RConn1 -- firing_circuit/RConn1

== system six_pulse_thyristor_based_rectifier/grid_line/six_pulse rectifier/BR2/ssc_thyristor_bridge/T3/Thyristor_3 ==
  Capacitor : fl_lib/Electrical/Electrical Elements/Capacitor  c=Csnubber_m F  r=Rsnubber_m Ohm  g=0 1/Ohm  i_specify=off  i_priority=None  i=0 A  i_nominal_specify=off  i_nominal_value=1  i_nominal_unit=A  v_specify=off  v_priority=None  v=0 V  v_nominal_specify=off  v_nominal_value=1  v_nominal_unit=V  vc_specify=off  vc_priority=High  vc=0 V  vc_nominal_specify=off  vc_nominal_value=1  vc_nominal_unit=V
  Current Sensor : fl_lib/Electrical/Electrical Sensors/Current Sensor
  Current Sensor1 : fl_lib/Electrical/Electrical Sensors/Current Sensor
  PS-Simulink Converter : nesl_utility/PS-Simulink Converter  PhysicalDomain=network_engine_domain  SubClassName=ps_output  LeftPortType=input  RightPortType=output  PseudoPeriodic=off  Frequencies=[]  VectorFormat=1-D array  Unit=A  AffineConversion=off
  PS-Simulink Converter1 : nesl_utility/PS-Simulink Converter  PhysicalDomain=network_engine_domain  SubClassName=ps_output  LeftPortType=input  RightPortType=output  PseudoPeriodic=off  Frequencies=[]  VectorFormat=1-D array  Unit=V  AffineConversion=off
  PS-Simulink Converter2 : nesl_utility/PS-Simulink Converter  PhysicalDomain=network_engine_domain  SubClassName=ps_output  LeftPortType=input  RightPortType=output  PseudoPeriodic=off  Frequencies=[]  VectorFormat=1-D array  Unit=A  AffineConversion=off
  Thyristor with Reverse Recovery (Lauritzen-Ma charge dynamics) : thyristor_rr_lib/Thyristor with Reverse Recovery (Lauritzen-Ma charge dynamics)  Vf=Vf_m V  Ron=Ron_m Ohm  Goff=Goff_m 1/Ohm  Vgt=Vgt_m V  Vth=forward_voltage_threshold_m V  Il=latching_current_m A  Ih=holding_current_m A  tau=carrier_lifetime_m s  Tm=charge_cross_time_constant_m s  Qth=residual_charge_threshold_m C  tq=circuit_commutated_turn_off_time_m s  i_specify=off  i_priority=None  i=0 A  i_nominal_specify=off  i_nominal_value=1  i_nominal_unit=A  v_specify=off  v_priority=None  v=0 V  v_nominal_specify=off  v_nominal_value=1  v_nominal_unit=V  qM_specify=off  qM_priority=High  qM=0 C  qM_nominal_specify=off  qM_nominal_value=1  qM_nominal_unit=C  on_specify=off  on_priority=None  on=0  toff_specify=off  toff_priority=None  toff=-1 s
  Voltage Sensor : fl_lib/Electrical/Electrical Sensors/Voltage Sensor
  K : PMIOPort  Side=Left
  G : PMIOPort  Port=2  Side=Right
  A : PMIOPort  Port=3  Side=Right
  tag scope: RC3_Id=scoped, TR3_Id=scoped, TR3_Ud=scoped
  wires:
  PS-Simulink Converter/1 -> [TR3_Id]
  PS-Simulink Converter2/1 -> [RC3_Id]
  PS-Simulink Converter1/1 -> [TR3_Ud]
  connections:
  Capacitor/LConn1 -- Voltage Sensor/RConn2 -- Thyristor with Reverse Recovery (Lauritzen-Ma charge dynamics)/RConn1 -- K/RConn1
  PS-Simulink Converter1/LConn1 -- Voltage Sensor/RConn1
  PS-Simulink Converter/LConn1 -- Current Sensor/RConn1
  Current Sensor1/RConn2 -- Capacitor/RConn1
  Voltage Sensor/LConn1 -- Current Sensor1/LConn1 -- Thyristor with Reverse Recovery (Lauritzen-Ma charge dynamics)/LConn1 -- Current Sensor/RConn2
  PS-Simulink Converter2/LConn1 -- Current Sensor1/RConn1
  Thyristor with Reverse Recovery (Lauritzen-Ma charge dynamics)/RConn2 -- G/RConn1
  A/RConn1 -- Current Sensor/LConn1

== system six_pulse_thyristor_based_rectifier/grid_line/six_pulse rectifier/BR2/ssc_thyristor_bridge/T3/firing3 ==
  Selector : Selector  InputPortWidth=6  IndexOptions=Index vector (dialog)  Indices=3  OutputSizes=1  RuntimeRangeChecks=off
  Simulink-PS Converter : nesl_utility/Simulink-PS Converter  PhysicalDomain=network_engine_domain  SubClassName=ps_input  LeftPortType=input  RightPortType=output  PseudoPeriodic=off  Frequencies=[]  NoiseDistribution=none  NoiseParameters=[]  Unit=V  AffineConversion=off  FilteringAndDerivatives=provide  SimscapeFilterOrder=1  InputFilterTimeConstant=0.001  UdotUserProvided=0
  firing_circuit : Subsystem
  strobe_gnr : Subsystem  Commented=through
  g+ : PMIOPort  Side=Right
  wires:
  strobe_gnr/1(out) -> Simulink-PS Converter/1
  [firing_cmds] -> Selector/1
  Selector/1 -> strobe_gnr/1(in)
  connections:
  Simulink-PS Converter/RConn1 -- firing_circuit/LConn1
  g+/RConn1 -- firing_circuit/RConn1

== system six_pulse_thyristor_based_rectifier/grid_line/six_pulse rectifier/BR2/ssc_thyristor_bridge/T4/Thyristor_4 ==
  Capacitor : fl_lib/Electrical/Electrical Elements/Capacitor  c=Csnubber_m F  r=Rsnubber_m Ohm  g=0 1/Ohm  i_specify=off  i_priority=None  i=0 A  i_nominal_specify=off  i_nominal_value=1  i_nominal_unit=A  v_specify=off  v_priority=None  v=0 V  v_nominal_specify=off  v_nominal_value=1  v_nominal_unit=V  vc_specify=off  vc_priority=High  vc=0 V  vc_nominal_specify=off  vc_nominal_value=1  vc_nominal_unit=V
  Current Sensor : fl_lib/Electrical/Electrical Sensors/Current Sensor
  Current Sensor1 : fl_lib/Electrical/Electrical Sensors/Current Sensor
  PS-Simulink Converter : nesl_utility/PS-Simulink Converter  PhysicalDomain=network_engine_domain  SubClassName=ps_output  LeftPortType=input  RightPortType=output  PseudoPeriodic=off  Frequencies=[]  VectorFormat=1-D array  Unit=A  AffineConversion=off
  PS-Simulink Converter1 : nesl_utility/PS-Simulink Converter  PhysicalDomain=network_engine_domain  SubClassName=ps_output  LeftPortType=input  RightPortType=output  PseudoPeriodic=off  Frequencies=[]  VectorFormat=1-D array  Unit=V  AffineConversion=off
  PS-Simulink Converter2 : nesl_utility/PS-Simulink Converter  PhysicalDomain=network_engine_domain  SubClassName=ps_output  LeftPortType=input  RightPortType=output  PseudoPeriodic=off  Frequencies=[]  VectorFormat=1-D array  Unit=A  AffineConversion=off
  Thyristor with Reverse Recovery (Lauritzen-Ma charge dynamics) : thyristor_rr_lib/Thyristor with Reverse Recovery (Lauritzen-Ma charge dynamics)  Vf=Vf_m V  Ron=Ron_m Ohm  Goff=Goff_m 1/Ohm  Vgt=Vgt_m V  Vth=forward_voltage_threshold_m V  Il=latching_current_m A  Ih=holding_current_m A  tau=carrier_lifetime_m s  Tm=charge_cross_time_constant_m s  Qth=residual_charge_threshold_m C  tq=circuit_commutated_turn_off_time_m s  i_specify=off  i_priority=None  i=0 A  i_nominal_specify=off  i_nominal_value=1  i_nominal_unit=A  v_specify=off  v_priority=None  v=0 V  v_nominal_specify=off  v_nominal_value=1  v_nominal_unit=V  qM_specify=off  qM_priority=High  qM=0 C  qM_nominal_specify=off  qM_nominal_value=1  qM_nominal_unit=C  on_specify=off  on_priority=None  on=0  toff_specify=off  toff_priority=None  toff=-1 s
  Voltage Sensor : fl_lib/Electrical/Electrical Sensors/Voltage Sensor
  K : PMIOPort  Side=Left
  G : PMIOPort  Port=2  Side=Right
  A : PMIOPort  Port=3  Side=Right
  tag scope: RC4_Id=scoped, TR4_Id=scoped, TR4_Ud=scoped
  wires:
  PS-Simulink Converter/1 -> [TR4_Id]
  PS-Simulink Converter2/1 -> [RC4_Id]
  PS-Simulink Converter1/1 -> [TR4_Ud]
  connections:
  Capacitor/LConn1 -- Voltage Sensor/RConn2 -- Thyristor with Reverse Recovery (Lauritzen-Ma charge dynamics)/RConn1 -- K/RConn1
  PS-Simulink Converter1/LConn1 -- Voltage Sensor/RConn1
  PS-Simulink Converter/LConn1 -- Current Sensor/RConn1
  Current Sensor1/RConn2 -- Capacitor/RConn1
  Voltage Sensor/LConn1 -- Current Sensor1/LConn1 -- Thyristor with Reverse Recovery (Lauritzen-Ma charge dynamics)/LConn1 -- Current Sensor/RConn2
  PS-Simulink Converter2/LConn1 -- Current Sensor1/RConn1
  Thyristor with Reverse Recovery (Lauritzen-Ma charge dynamics)/RConn2 -- G/RConn1
  A/RConn1 -- Current Sensor/LConn1

== system six_pulse_thyristor_based_rectifier/grid_line/six_pulse rectifier/BR2/ssc_thyristor_bridge/T4/firing4 ==
  Selector : Selector  InputPortWidth=6  IndexOptions=Index vector (dialog)  Indices=4  OutputSizes=1  RuntimeRangeChecks=off
  Simulink-PS Converter : nesl_utility/Simulink-PS Converter  PhysicalDomain=network_engine_domain  SubClassName=ps_input  LeftPortType=input  RightPortType=output  PseudoPeriodic=off  Frequencies=[]  NoiseDistribution=none  NoiseParameters=[]  Unit=V  AffineConversion=off  FilteringAndDerivatives=provide  SimscapeFilterOrder=1  InputFilterTimeConstant=0.001  UdotUserProvided=0
  firing_circuit : Subsystem
  strobe_gnr : Subsystem  Commented=through
  g+ : PMIOPort  Side=Right
  wires:
  strobe_gnr/1(out) -> Simulink-PS Converter/1
  Selector/1 -> strobe_gnr/1(in)
  [firing_cmds] -> Selector/1
  connections:
  Simulink-PS Converter/RConn1 -- firing_circuit/LConn1
  g+/RConn1 -- firing_circuit/RConn1

== system six_pulse_thyristor_based_rectifier/grid_line/six_pulse rectifier/BR2/ssc_thyristor_bridge/T5/Thyristor_5 ==
  Capacitor : fl_lib/Electrical/Electrical Elements/Capacitor  c=Csnubber_m F  r=Rsnubber_m Ohm  g=0 1/Ohm  i_specify=off  i_priority=None  i=0 A  i_nominal_specify=off  i_nominal_value=1  i_nominal_unit=A  v_specify=off  v_priority=None  v=0 V  v_nominal_specify=off  v_nominal_value=1  v_nominal_unit=V  vc_specify=off  vc_priority=High  vc=0 V  vc_nominal_specify=off  vc_nominal_value=1  vc_nominal_unit=V
  Current Sensor : fl_lib/Electrical/Electrical Sensors/Current Sensor
  Current Sensor1 : fl_lib/Electrical/Electrical Sensors/Current Sensor
  PS-Simulink Converter : nesl_utility/PS-Simulink Converter  PhysicalDomain=network_engine_domain  SubClassName=ps_output  LeftPortType=input  RightPortType=output  PseudoPeriodic=off  Frequencies=[]  VectorFormat=1-D array  Unit=A  AffineConversion=off
  PS-Simulink Converter1 : nesl_utility/PS-Simulink Converter  PhysicalDomain=network_engine_domain  SubClassName=ps_output  LeftPortType=input  RightPortType=output  PseudoPeriodic=off  Frequencies=[]  VectorFormat=1-D array  Unit=V  AffineConversion=off
  PS-Simulink Converter2 : nesl_utility/PS-Simulink Converter  PhysicalDomain=network_engine_domain  SubClassName=ps_output  LeftPortType=input  RightPortType=output  PseudoPeriodic=off  Frequencies=[]  VectorFormat=1-D array  Unit=A  AffineConversion=off
  Thyristor with Reverse Recovery (Lauritzen-Ma charge dynamics) : thyristor_rr_lib/Thyristor with Reverse Recovery (Lauritzen-Ma charge dynamics)  Vf=Vf_m V  Ron=Ron_m Ohm  Goff=Goff_m 1/Ohm  Vgt=Vgt_m V  Vth=forward_voltage_threshold_m V  Il=latching_current_m A  Ih=holding_current_m A  tau=carrier_lifetime_m s  Tm=charge_cross_time_constant_m s  Qth=residual_charge_threshold_m C  tq=circuit_commutated_turn_off_time_m s  i_specify=off  i_priority=None  i=0 A  i_nominal_specify=off  i_nominal_value=1  i_nominal_unit=A  v_specify=off  v_priority=None  v=0 V  v_nominal_specify=off  v_nominal_value=1  v_nominal_unit=V  qM_specify=off  qM_priority=High  qM=0 C  qM_nominal_specify=off  qM_nominal_value=1  qM_nominal_unit=C  on_specify=off  on_priority=None  on=0  toff_specify=off  toff_priority=None  toff=-1 s
  Voltage Sensor : fl_lib/Electrical/Electrical Sensors/Voltage Sensor
  K : PMIOPort  Side=Left
  G : PMIOPort  Port=2  Side=Right
  A : PMIOPort  Port=3  Side=Right
  tag scope: RC5_Id=scoped, TR5_Id=scoped, TR5_Ud=scoped
  wires:
  PS-Simulink Converter/1 -> [TR5_Id]
  PS-Simulink Converter2/1 -> [RC5_Id]
  PS-Simulink Converter1/1 -> [TR5_Ud]
  connections:
  Capacitor/LConn1 -- Voltage Sensor/RConn2 -- Thyristor with Reverse Recovery (Lauritzen-Ma charge dynamics)/RConn1 -- K/RConn1
  PS-Simulink Converter1/LConn1 -- Voltage Sensor/RConn1
  PS-Simulink Converter/LConn1 -- Current Sensor/RConn1
  Current Sensor1/RConn2 -- Capacitor/RConn1
  Voltage Sensor/LConn1 -- Current Sensor1/LConn1 -- Thyristor with Reverse Recovery (Lauritzen-Ma charge dynamics)/LConn1 -- Current Sensor/RConn2
  PS-Simulink Converter2/LConn1 -- Current Sensor1/RConn1
  Thyristor with Reverse Recovery (Lauritzen-Ma charge dynamics)/RConn2 -- G/RConn1
  A/RConn1 -- Current Sensor/LConn1
